simulink model "ATOM_simple_planning_simulator"  (R2026a)
settings: Solver=ode4  StopTime=100  FixedStep=0.01
StopFcn:
  | % Put every new figure in the same MATLAB Figures window as a docked tab.
  | set(groot, 'defaultFigureWindowStyle', 'docked');
  | 
  | if exist('costmap_active', 'var') && ...
  |     exist('vehicle', 'var') && ...
  |     exist('parking_path', 'var') && ...
  |     ~isempty(parking_path)
  | 
  |      plotPlan(costmap_active, vehicle, parking_path);
  | 
  |  else
  | 
  |      warning('No valid parking path is available for plotting.');
  | 
  |  end
  | 
  |  PlotControllerReferences( ...
  |      out.controller_reference_log);
  | 
  |  PlotControllerTracking( ...
  |      out.controller_tracking_log);
  | 
model workspace (MAT data in the model file):
  vehicle : object (value not decoded)
symbols that are objects in the model workspace (value not decoded): vehicle
undefined symbols (not defined in the file): delta_f_LUT, gain4WS_LUT, k_ref_LUT, kappa_gain_BP, Ki, Kp, lateral, longitudinal, planning_validator, rr_gain_BP, rr_LUT, stanley, velocity_smoother
libraries: slpidlib x1
(part 3 of 8)

== matlab function ATOM_simple_planning_simulator/time_parameterization2/Time parameterization ==
  data: trajectory_in input Bus: TrajectoryDataBus size=1; reference_out output Bus: ParkingReferenceBus size=1; steer_rate_limit input
function reference_out = timeParameterization( ...
    trajectory_in,steer_rate_limit)
%#codegen
%
% Convert the 100-point spatial parking trajectory into a nominal
% time-parameterized reference trajectory.

N = 100;

%% Extract the smoothed trajectory

x_ref = trajectory_in.pose.position.x;
y_ref = trajectory_in.pose.position.y;

qz = trajectory_in.pose.orientation.qz;
qw = trajectory_in.pose.orientation.qw;

v_ref = trajectory_in.longitudinal_velocity_mps;
a_ref = trajectory_in.acceleration_mps2;

df_plan = trajectory_in.front_wheel_angle_rad;
dr_plan = trajectory_in.rear_wheel_angle_rad;

rear_angle = trajectory_in.rear_wheel_angle_rad;

%% Convert quaternion to continuous body-heading reference

psi_ref = zeros(N,1);

psi_ref(1) = 2.0*atan2(qz(1),qw(1));

for k = 2:N

    raw_heading = 2.0*atan2(qz(k),qw(k));

    heading_change = raw_heading-psi_ref(k-1);

    psi_ref(k) = ...
        raw_heading-2.0*pi*round(heading_change/(2.0*pi));
end

%% Calculate distance and nominal time

s_ref = zeros(N,1);
t_ref = zeros(N,1);

for k = 1:N-1

    dx = x_ref(k+1)-x_ref(k);
    dy = y_ref(k+1)-y_ref(k);

    ds = hypot(dx,dy);

    s_ref(k+1) = s_ref(k)+ds;

    % Convert signed body-longitudinal velocity to positive rear-axle
    % path speed.
    path_speed_current = ...
        abs(v_ref(k))/max(cos(rear_angle(k)),0.1);

    path_speed_next = ...
        abs(v_ref(k+1))/max(cos(rear_angle(k+1)),0.1);

    speed_sum = path_speed_current+path_speed_next;

    if ds <= 1e-9

        dt = 0.0;

    elseif speed_sum > 1e-6

        % ds = 0.5*(v_current+v_next)*dt
        dt = 2.0*ds/speed_sum;

    else

        % Protect against an interval whose two endpoint speeds are zero.
        fallback_path_speed = 0.05;

        dt = ds/fallback_path_speed;
    end

    t_ref(k+1) = t_ref(k)+dt;
end
N = numel(t_ref);

df_nom = zeros(size(df_plan));
dr_nom = zeros(size(dr_plan));

% Start from the planner's first steering configuration.
df_nom(1) = df_plan(1);
dr_nom(1) = dr_plan(1);

for i = 2:N

    dt = max(t_ref(i)-t_ref(i-1),0.0);
    maximum_change = steer_rate_limit*dt;

    front_difference = df_plan(i)-df_nom(i-1);
    rear_difference  = dr_plan(i)-dr_nom(i-1);

    front_change = max( ...
        -maximum_change, ...
        min(maximum_change,front_difference));

    rear_change = max( ...
        -maximum_change, ...
        min(maximum_change,rear_difference));

    df_nom(i) = df_nom(i-1)+front_change;
    dr_nom(i) = dr_nom(i-1)+rear_change;

end

reference_out.t_ref   = t_ref;
reference_out.s_ref   = s_ref;
reference_out.x_ref   = x_ref;
reference_out.y_ref   = y_ref;
reference_out.psi_ref = psi_ref;
reference_out.v_ref   = v_ref;
reference_out.a_ref   = a_ref;
% Temporary pass-through. The next step will make these rate-feasible.
reference_out.df_nom = df_nom;
reference_out.dr_nom = dr_nom;
end

== matlab function ATOM_simple_planning_simulator/Plot demanded trajectory ==
  data: traj input
function plotTrajectory(traj)

persistent hTraj hArrow


x = traj.pose.position.x;
y = traj.pose.position.y;

yaw = zeros(length(x),1);


for i=1:length(x)

    yaw(i)=2*atan2(...
        traj.pose.orientation.qz(i),...
        traj.pose.orientation.qw(i));

end


if isempty(hTraj)

    figure(2)
    clf
    hold on
    grid on
    axis equal

    hTraj=plot(x,y,'b','LineWidth',2);


    step=5;

    hArrow=quiver(...
        x(1:step:end),...
        y(1:step:end),...
        cos(yaw(1:step:end)),...
        sin(yaw(1:step:end)),...
        0.5,...
        'r');

else

    set(hTraj,...
        'XData',x,...
        'YData',y);

end


drawnow limitrate

end

== matlab function ATOM_simple_planning_simulator/velocity_smoother_node/ApplySteeringRateLimit - velocity_smoother_node/ApplyPreProcess ==
  data: input input Bus: TrajectoryDataBus; use_resempling input boolean; output output Bus: TrajectoryDataBus; points_interval input double
function output = applyPreProcess(input, use_resempling, points_interval)

% ApplyPreProcess
%
% This function reproduces the first stage of Autoware
% SmootherBase::applyPreProcess().
%
% In Autoware, when resampling is enabled, the input trajectory
% is interpolated with a constant spatial interval.
%
% In this Simulink implementation the resampling stage is omitted
% (use_resempling == false)
% The original trajectory points are directly forwarded to the next block.
%

output = input;

end

== matlab function ATOM_simple_planning_simulator/velocity_smoother_node/ApplySteeringRateLimit - velocity_smoother_node/Step1: Calculate curvature assuming the trajectory points interval is constant./CalcTrajectoryCurvature ==
  data: trajectory input Bus: TrajectoryDataBus; curvature output; idx_dist input
function curvature = ComputeTrajectoryCurvature( ...
    trajectory, ...
    idx_dist)

% ComputeTrajectoryCurvature
%
% Computes the geometric curvature of a trajectory using a three-point
% circle fitting method.
%
% This function reproduces the behavior of:
%
% autoware_motion_utils::calcTrajectoryCurvatureFrom3Points()
%
% used inside:
%
% autoware_velocity_smoother
%
% In the original Autoware implementation, the curvature computation:
%
%   curvature = calc_curvature(p0,p1,p2)
%
% is protected by a C++ try/catch block. If the circle fitting fails
% (for example due to degenerate geometry), Autoware keeps the previous
% curvature value.
%
% MATLAB/Simulink code generation does not support try/catch constructs.
% Therefore this implementation assumes that calc_curvature() is robust
% and handles degenerate cases internally.
%
% Inputs
% -------
% trajectory : struct
%
%   MATLAB representation of Autoware TrajectoryPoints.
%
%   Autoware source:
%
%   autoware_motion_utils/src/trajectory/conversion.cpp
%
%   converts:
%
%       autoware_planning_msgs::msg::Trajectory
%
%   into:
%
%       std::vector<autoware_planning_msgs::msg::TrajectoryPoint>
%
%   via:
%
    % std::vector<autoware_planning_msgs::msg::TrajectoryPoint> convertToTrajectoryPointArray(
    % const autoware_planning_msgs::msg::Trajectory & trajectory)
    % {
    %     std::vector<autoware_planning_msgs::msg::TrajectoryPoint> output(trajectory.points.size());
    %     std::copy(trajectory.points.begin(), trajectory.points.end(), output.begin());
    %     return output;
    % }
%
%
%
%   Each trajectory point contains:
%
%       geometry_msgs/msg/Point pose.position
%
%   with:
%
%       x, y, z
%
%   MATLAB representation:
%
%       trajectory.pose.position.x
%       trajectory.pose.position.y
%       trajectory.pose.position.z
%
%
% idx_dist : scalar
%
%   Number of trajectory samples used as offset for the three-point
%   curvature estimation.
%
%   In Autoware:
%
%       idx_dist =
%       max(floor(curvature_calculation_distance / points_interval),1)
%
%
% Output
% -------
% curvature : Nx1 vector
%
%   Estimated trajectory curvature [1/m].

num_points = length(trajectory.pose.position.x);


%% Not enough trajectory points

% Autoware:
%
% if (trajectory.size() < 3)
% {
%     return vector filled with zeros;
% }

if num_points < 3
    curvature = zeros(num_points,1);
    return;
end


%% Limit idx_dist according to trajectory size

% Autoware:
%
% max_idx_dist =
% floor((trajectory.size()-1)/2)
%
% idx_dist =
% max(1,min(idx_dist,max_idx_dist))

max_idx_dist = floor((num_points-1)/2);

idx_dist = max(1,min(idx_dist,max_idx_dist));


%% Initialize curvature vector

% Autoware:
%
% std::vector<double> k_arr(trajectory.size(),0.0);

curvature = zeros(num_points,1);


%% Three-point curvature estimation

% Autoware:
%
% for (size_t i = 1; i + 1 < trajectory.size(); i++)

% MATLAB indexing:
%
% i = 2 ... N-1

for i = 2:num_points-1


    % Select the three points:
    %
    % p0 : idx_dist samples before
    % p1 : current trajectory point
    % p2 : idx_dist samples after
    %
    % Equivalent to Autoware:
    %
    % p0 = get_point(
    %       trajectory.at(i - min(idx_dist,i)))
    %
    % p1 = get_point(
    %       trajectory.at(i))
    %
    % p2 = get_point(
    %       trajectory.at(
    %       i + min(idx_dist,size-i-1)))


    idx_prev = i - min(idx_dist,i-1);

    idx_curr = i;

    idx_next = i + min(idx_dist,num_points-i);


    % geometry_msgs/msg/Point:
    %
    % float64 x
    % float64 y
    % float64 z

    p0 = [
        trajectory.pose.position.x(idx_prev), ...
        trajectory.pose.position.y(idx_prev), ...
        trajectory.pose.position.z(idx_prev)
        ];

    p1 = [
        trajectory.pose.position.x(idx_curr), ...
        trajectory.pose.position.y(idx_curr), ...
        trajectory.pose.position.z(idx_curr)
        ];

    p2 = [
        trajectory.pose.position.x(idx_next), ...
        trajectory.pose.position.y(idx_next), ...
        trajectory.pose.position.z(idx_next)
        ];


    %% Compute curvature

    % Autoware:
    %
    % try
    % {
    %     curvature = calc_curvature(p0,p1,p2);
    % }
    %
    % catch(...)
    % {
    %     curvature = previous curvature;
    % }
    %
    % try/catch removed because unsupported by Simulink Coder.

    curvature(i) = calc_curvature(p0,p1,p2);


end


%% Boundary curvature completion

% Autoware:
%
% k_arr.at(0) = k_arr.at(1);
% k_arr.back() = k_arr.at(size-2);

curvature(1) = curvature(2);

curvature(end) = curvature(end-1);


end

== matlab function ATOM_simple_planning_simulator/velocity_smoother_node/ApplySteeringRateLimit - velocity_smoother_node/Step4: Limit velocity by steer rate./ApplySteeringRateVelocityLimit ==
  data: steer_rate_velocity_ratio_limits input; curvature input; steer_rate_ratio input; curvature_threshold input; min_curve_velocity input; velocity_thresholds input; steering_angle_rate_limits input; trajectory input Bus: TrajectoryDataBus; trajectory output
function trajectory = ApplySteeringRateVelocityLimit( ...
    steer_rate_velocity_ratio_limits, ...
    curvature, ...
    steer_rate_ratio, ...
    curvature_threshold, ...
    min_curve_velocity, ...
    velocity_thresholds, ...
    steering_angle_rate_limits, ...
    trajectory)

% ApplySteeringRateVelocityLimit
%
% Applies the steering-rate velocity constraint to the trajectory.
%
% Equivalent to Step 4 of:
%
%   SmootherBase::applySteeringRateLimit()
%
% in Autoware.
%
%
% The steering rate itself does not directly modify the steering angles.
% Instead, it generates a local maximum admissible velocity.
%
% Whenever the current trajectory speed exceeds this limit,
% the trajectory longitudinal velocity is reduced.
%
%
% This algorithm is identical for both 2WS and 4WS.
%
% The only difference is how steer_rate_ratio has been computed.
%
%
% In C++, the following reference:
%
%   auto & velocity =
%       output.at(i+k).longitudinal_velocity_mps;
%
% directly modifies the trajectory.
%
% MATLAB has no equivalent reference semantics, therefore the trajectory
% structure is explicitly updated.



N = length(trajectory.longitudinal_velocity_mps);


for i = 1:N-1

    %% Ignore almost straight segments

    if abs(curvature(i)) < curvature_threshold
        continue
    end


    %% Mean velocity

    mean_velocity = ...
        ( ...
        trajectory.longitudinal_velocity_mps(i) + ...
        trajectory.longitudinal_velocity_mps(i+1) ...
        ) / 2;


    %% Local steering-rate velocity limit

    local_velocity_limit = ...
        ComputeVelocityLimitFromSteerRate( ...
        steer_rate_ratio(i), ...
        steer_rate_velocity_ratio_limits, ...
        velocity_thresholds, ...
        steering_angle_rate_limits);

    %% If the following condition is true, do nothing and pass to the next iteration

    if mean_velocity < local_velocity_limit
        continue
    end


    %% Update the two neighbouring trajectory points

    % Equivalent in C++ to:
    % for (size_t k = 0; k < 2; k++) {
    %     auto & velocity = output.at(i+k).longitudinal_velocity_mps;
    % 
    %     const float target_velocity =
    %     std::max(
    %     min_curve_velocity,
    %     std::min(
    %     local_velocity_limit,
    %     velocity * (local_velocity_limit / mean_vel)));
    % 
    %     velocity = std::min(velocity,target_velocity);
    %     }

    for k = 0:1

        idx = i + k;

        velocity = ...
            trajectory.longitudinal_velocity_mps(idx);


        target_velocity = max( ...
            min_curve_velocity, ...
            min( ...
                local_velocity_limit, ...
                velocity * ...
                (local_velocity_limit / mean_velocity)));


        trajectory.longitudinal_velocity_mps(idx) = ...
            min(velocity, target_velocity);

    end

end

end

== matlab function ATOM_simple_planning_simulator/velocity_smoother_node/ApplySteeringRateLimit - velocity_smoother_node/Step2: Calculate steer rate for each trajectory point/ComputeSteeringRate4WS ==
  data: trajectory input Bus: TrajectoryDataBus; curvature input; veh input; steer_rate_velocity_ratio_arr output; points_interval input; output output Bus: TrajectoryDataBus; k_ref_LUT input; rr_LUT input; delta_f_LUT input
function [steer_rate_velocity_ratio_arr, output] = ComputeSteeringRateAngle4WS(trajectory, ...
    curvature, veh, ...
    points_interval, ...
    k_ref_LUT, rr_LUT, delta_f_LUT)


% ComputeSteeringRateAngle4WS
%
% Computes steering angle rate ratio for 4WS.
%
% Equivalent to Autoware:
%
% steer_rate_velocity_ratio_arr
%
%
% The returned value represents:
%
%       steering_angle_difference / distance
%
%
% For 4WS:
%
% front and rear steering rates are computed.
%
% The maximum steering variation is used as constraint.


N = length(curvature);

rr = zeros(N,1);
front_angle = zeros(N,1);
rear_angle  = zeros(N,1);


%% Compute steering angles

for i = 1:N
    
    if curvature(i) > max(k_ref_LUT)
        rr(i) = -1;
        front_angle(i) = 0.7;
        rear_angle(i) = -0.7;
    else                                                         % Modified for 4WS
        rr(i) = interp1(k_ref_LUT, rr_LUT, curvature(i));
        front_angle(i) = interp1(k_ref_LUT, delta_f_LUT, curvature(i));
        rear_angle(i) = rr(i) * front_angle(i);      
    end
end

% This is a collateral effect of (&) in C++ when (considering in original
% Autoware):
%
% auto & steer_front = output.at(i + 1).front_wheel_angle_rad;
% auto & steer_back = output.at(i).front_wheel_angle_rad;
% 
% // calculate the just 2 steering angle
% steer_front = std::atan(base_param_.wheel_base * curvature_v.at(i + 1));
% steer_back = std::atan(base_param_.wheel_base * curvature_v.at(i));
% Indeed, updating steer_front we popolate also output.at(i + 1).front_wheel_angle_rad, 
% and so the output topic is populated (but it's just a collateral effect, front_wheel_angle_rad 
% and rear_wheel_angle_rad contents are not important for Control module.

trajectory.front_wheel_angle_rad = front_angle;
trajectory.rear_wheel_angle_rad  = rear_angle;

%% Compute steering rate

steer_rate_velocity_ratio_arr = zeros(N,1);


for i = 1:N-1


    % auto & steer_front = output.at(i + 1).front_wheel_angle_rad;
    % auto & steer_back = output.at(i).front_wheel_angle_rad;
    % const auto steering_diff = std::fabs(steer_front - steer_back);
    front_diff = abs( ...
        front_angle(i+1)-front_angle(i));


    rear_diff = abs( ...
        rear_angle(i+1)-rear_angle(i));


    steering_diff = max( ...                                    % Modified for 4WS --> conservative solution
        front_diff,...
        rear_diff);

    % eps avoids division by zero:
    eps = 2.220446049250313e-16;

    steer_rate_velocity_ratio_arr(i)= ...
        steering_diff/(points_interval+eps);


end


steer_rate_velocity_ratio_arr(end)= ...
    steer_rate_velocity_ratio_arr(end-1);


% Output topic now presents front_wheel_angle_rad and rear_wheel_angle_rad
% populated
output = trajectory;


end

== matlab function ATOM_simple_planning_simulator/velocity_smoother_node/ApplySteeringRateLimit - velocity_smoother_node/Step3: Remove noise by mean filter/MeanFilterSteeringRateRato ==
  data: steer_rate_ratio input; steer_rate_velocity_ratio_arr output
function steer_rate_velocity_ratio_arr = MeanFilterSteeringRateRatio( ...
    steer_rate_ratio)

% MeanFilterSteeringRateRatio
%
% Applies the same moving-average filter used by Autoware on the steering
% rate ratio.
%
% Equivalent to Step 3 inside:
%
%   SmootherBase::applySteeringRateLimit()
%
% in:
%
%   autoware_velocity_smoother
%
%
% Original C++ implementation:
%
% for (size_t i = 1; i < steer_rate_velocity_ratio_arr.size() - 1; i++) {
%
%   steer_rate_velocity_ratio_arr.at(i) =
%     (steer_rate_velocity_ratio_arr.at(i-1) +
%      steer_rate_velocity_ratio_arr.at(i)   +
%      steer_rate_velocity_ratio_arr.at(i+1))
%      / 3.0;
%
% }
%
%
% Notes
% -----
%
% The filter is performed in-place, exactly as in Autoware.
%
% Consequently, when computing sample i, the previous sample
% (i-1) has already been filtered, while the next sample (i+1)
% is still the original one.
%
% This behaviour is intentionally preserved to remain identical
% to the C++ implementation.


N = length(steer_rate_ratio);

steer_rate_velocity_ratio_arr = zeros(N,1);

for i = 2:N-1

    steer_rate_velocity_ratio_arr(i) = ...
        ( ...
        steer_rate_ratio(i-1) + ...
        steer_rate_ratio(i)   + ...
        steer_rate_ratio(i+1) ...
        ) / 3.0;

end


end

== matlab function ATOM_simple_planning_simulator/velocity_smoother_node/ApplySteeringRateLimit - velocity_smoother_node/ComputePointsInterval ==
  data: input_points_interval input; vel_smoother input; use_resampling input; points_interval output
function points_interval = computePointsInterval(input_points_interval, ...
    vel_smoother, use_resampling)

% Compute the trajectory points interval used for preprocessing.
%
% If resampling is enabled, a constant spatial interval is imposed.
% Otherwise, the original trajectory point spacing is preserved.

sample_ds = vel_smoother(3,1);

if use_resampling

    points_interval = sample_ds;

else

    points_interval = input_points_interval;

end

end

== matlab function ATOM_simple_planning_simulator/velocity_smoother_node/ApplySteeringRateLimit - velocity_smoother_node/ComputeIdxDist ==
  data: points_interval input; idx_dist output; vel_smoother input
function idx_dist = ComputeIdxDist( ...
    points_interval, ...
    vel_smoother)

% ComputeIdxDist
%
% Computes the point offset used for trajectory curvature estimation.
%
% The curvature is evaluated using three trajectory points separated by a
% fixed physical distance. Since the trajectory is sampled with a constant
% spatial interval (points_interval), this function converts the desired
% curvature calculation distance into the corresponding point index offset.
%
% In other words, idx_dist represents the number of trajectory points
% corresponding to the specified curvature calculation distance.
%
% Equivalent to the Autoware implementation:
%
% idx_dist = max(int(curvature_calculation_distance / points_interval), 1);

curvature_calculation_distance = vel_smoother(1);

idx_dist = max( ...
    floor(curvature_calculation_distance / points_interval), ...
    1);

== matlab function ATOM_simple_planning_simulator/velocity_smoother_node/ApplySteeringRateLimit - velocity_smoother_node/PlotTrajectoryCurvature ==
  data: trajectory input; curvature input
function PlotTrajectoryCurvature(trajectory, curvature)

% PlotTrajectoryCurvature
%
% Visualizes the trajectory curvature computed by:
%
%   ComputeTrajectoryCurvature()
%
% Equivalent to inspecting:
%
%   std::vector<double> k_arr
%
% generated inside:
%
%   autoware_motion_utils::calcTrajectoryCurvatureFrom3Points()
%
%
% Inputs
% -------
%
% trajectory:
%   MATLAB representation of Autoware TrajectoryPoints:
%
%       trajectory.pose.position.x
%       trajectory.pose.position.y
%
%
% curvature:
%   Nx1 signed curvature vector [1/m].
%
%   Positive curvature  -> left turn
%   Negative curvature  -> right turn


persistent hCurvature
persistent hTraj


%% Extract trajectory position

x = trajectory.pose.position.x;
y = trajectory.pose.position.y;


%% Check dimensions

if length(curvature) ~= length(x)

    error("Curvature vector length does not match trajectory length.");

end


%% Curvature profile

if isempty(hCurvature) 

    figure(3)
    clf

    hold on
    grid on

    hCurvature = plot( ...
        curvature, ...
        'LineWidth',1.5);


    xlabel("Trajectory point index");
    ylabel("Curvature [1/m]");

    title("Curvature profile");


else

    set(hCurvature,...
        'YData',curvature);

end



%% XY trajectory colored by curvature

if isempty(hTraj) 

    figure(4)
    clf

    hold on
    grid on
    axis equal


    hTraj = scatter( ...
        x, ...
        y, ...
        25, ...
        curvature, ...
        'filled');


    xlabel("x [m]");
    ylabel("y [m]");

    title("Trajectory curvature map");


    cb = colorbar;
    ylabel(cb,'Curvature [1/m]');


else

    set(hTraj,...
        'XData',x,...
        'YData',y,...
        'CData',curvature);

end


drawnow limitrate


end

== matlab function ATOM_simple_planning_simulator/velocity_smoother_node/ApplySteeringRateLimit - velocity_smoother_node/ComputeSteerRateVelocityRatioLimits ==
  data: velocity_thresholds input; steer_rate_velocity_ratio_limits output; steering_angle_rate_limits input
function steer_rate_velocity_ratio_limits = ...
    ComputeSteerRateVelocityRatioLimits( ...
    velocity_thresholds, ...
    steering_angle_rate_limits)

% ComputeSteerRateVelocityRatioLimits
%
% MATLAB equivalent of:
%
%   SmootherBase::computeSteerRateVelocityRatioLimits()
%
% in Autoware.
%
% It computes the steering-rate / velocity ratio limits used later by
% ComputeVelocityLimitFromSteerRate().
%
%
% Equivalent C++:
%
% return computeRatioLimits<double>(
%     velocity_thresholds,
%     steering_angle_rate_limits,
%     compute_steer_rate_ratio);
%
%
% Inputs
% -------
%
% velocity_thresholds
%       Velocity breakpoints [m/s]
%
% steering_angle_rate_limits
%       Maximum steering rate [deg/s]
%
%
% Output
% ------
%
% steer_rate_velocity_ratio_limits
%
% Nx2 matrix equivalent to:
%
% std::vector<std::pair<double,double>>
%
% Each row contains:
%
%   [ratio_lower , ratio_upper]
%
% corresponding to one velocity interval.


epsilon = 1e-5;

N = length(velocity_thresholds);

steer_rate_velocity_ratio_limits = zeros(N+1,2);


%% Compute ratio limits

for i = 1:N

    rate_deg = steering_angle_rate_limits(i);

    vi = velocity_thresholds(i);

    if i == 1
        vi_prev = 0.0;
    else
        vi_prev = velocity_thresholds(i-1);
    end

    steer_rate_velocity_ratio_limits(i,1) = ...
        deg2rad(rate_deg)/(vi_prev + epsilon);

    steer_rate_velocity_ratio_limits(i,2) = ...
        deg2rad(rate_deg)/(vi + epsilon);

end


%% Last interval

v_max = velocity_thresholds(end);

steer_rate_velocity_ratio_limits(end,1) = ...
    deg2rad(steering_angle_rate_limits(end)) / ...
    (v_max + epsilon);

steer_rate_velocity_ratio_limits(end,2) = 0.0;

end

== matlab function ATOM_simple_planning_simulator/velocity_smoother_node/MATLAB Function ==
  data: trajectory_input input; trajectory_output input; curvature input
function PlotSteeringRateVelocityLimit( ...
    trajectory_input, ...
    trajectory_output, ...
    curvature)

% PlotSteeringRateVelocityLimit
%
% Visualizes the velocity modification produced by the steering-rate
% velocity constraint.
%
% Equivalent to inspecting the difference between:
%
%   input.longitudinal_velocity_mps
%
% and:
%
%   output.longitudinal_velocity_mps
%
% after:
%
%   SmootherBase::applySteeringRateLimit()
%
% in Autoware.
%
%
% The steering-rate filter does not modify the trajectory geometry.
% It only reduces longitudinal velocity where the steering rate
% constraint is violated.
%
%
% Inputs
% -------
%
% trajectory_input:
%       Trajectory before ApplySteeringRateVelocityLimit()
%
%       Required fields:
%           trajectory.longitudinal_velocity_mps
%
%
% trajectory_output:
%       Trajectory after ApplySteeringRateVelocityLimit()
%
%       Required fields:
%           trajectory.longitudinal_velocity_mps
%
%
% curvature:
%       trajectory curvature [1/m]
%
%       Used only for visualization of curved regions.
%
%
% Output
% -------
%
% None
%
% Generates diagnostic plots:
%
%   - velocity before/after steering-rate constraint
%   - velocity reduction
%   - curvature profile


%% Extract velocities

vel_in = trajectory_input.longitudinal_velocity_mps;
vel_out = trajectory_output.longitudinal_velocity_mps;


N = length(vel_in);


if length(vel_out) ~= N
    error("Input and output trajectories have different lengths.");
end


%% Velocity variation

velocity_delta = vel_out - vel_in;


%% Plot velocity profile

persistent hVelIn hVelOut hCurvature hVelDelta1 hVelDelta2


if isempty(hVelIn)

    figure(5)
    hold on
    grid on

    hVelIn = plot( ...
        vel_in,...
        'LineWidth',1.5,...
        'DisplayName',"Input velocity");
    
    hVelOut = plot( ...
        vel_out,...
        '--',...
        'LineWidth',1.5,...
        'DisplayName',"After steering-rate limit");


    xlabel("Trajectory point index");
    ylabel("Longitudinal velocity [m/s]");
    
    title("Steering-rate velocity limitation");
    
    legend("Location","best");

else
    
    set(hVelIn, ...
        'YData', vel_in);
    
    set(hVelOut, ...
        'YData', vel_out);
end

%% Plot velocity reduction


if isempty(hVelDelta1)

    figure(6)
    hold on
    grid on

    hVelDelta1 = plot( ...
        velocity_delta,...
        'LineWidth',1.5);
    
    
    yline(0);
    
    
    xlabel("Trajectory point index");
    ylabel("\Delta velocity [m/s]");
    
    
    title("Velocity modification due to steering-rate constraint");

else

    set(hVelDelta1, ...
        'YData', velocity_delta);


end

drawnow limitrate

end

== matlab function ATOM_simple_planning_simulator/Lane Follower Scenario/Demanded trajectory generation: Sinusoid 50m wavelength/Trajectory Generator: sinusoid ==
  data: x output; y output; z output; qx output; qy output; qz output; qw output; longitudinal_velocity_mps output; lateral_velocity_mps output; acceleration_mps2 output; heading_rate_rps output; front_wheel_angle_rad output; rear_wheel_angle_rad output
function [x,y,z,qx,qy,qz,qw,...
    longitudinal_velocity_mps,...
    lateral_velocity_mps,...
    acceleration_mps2,...
    heading_rate_rps,...
    front_wheel_angle_rad,...
    rear_wheel_angle_rad] = trajectoryGenerator

N = 100;

L = 100;                % trajectory length [m]
A = 5;                  % sinusoid amplitude [m]

x = linspace(0,L,N)';
y = A*sin(2*pi*x/50);      % wavelength = 50 m

z = zeros(N,1);

qx = zeros(N,1);
qy = zeros(N,1);
qz = zeros(N,1);
qw = zeros(N,1);

longitudinal_velocity_mps = (8/3.6)*ones(N,1);

lateral_velocity_mps = zeros(N,1);
acceleration_mps2    = zeros(N,1);
heading_rate_rps     = zeros(N,1);

front_wheel_angle_rad = zeros(N,1);
rear_wheel_angle_rad  = zeros(N,1);

%% Orientation

dy = gradient(y,x);

yaw = atan(dy);

qz = sin(yaw/2);
qw = cos(yaw/2);

end

== matlab function ATOM_simple_planning_simulator/Lane Follower Scenario/Demanded trajectory generation: 90° left turn/Trajectory Generator: 90° left turn ==
  data: x output; y output; z output; qx output; qy output; qz output; qw output; longitudinal_velocity_mps output; lateral_velocity_mps output; acceleration_mps2 output; heading_rate_rps output; front_wheel_angle_rad output; rear_wheel_angle_rad output
function [x,y,z,qx,qy,qz,qw,...
          longitudinal_velocity_mps,...
          lateral_velocity_mps,...
          acceleration_mps2,...
          heading_rate_rps,...
          front_wheel_angle_rad,...
          rear_wheel_angle_rad] = trajectoryGenerator

N = 100;

%% Geometry

R = 10;              % curve radius [m]

N1 = 30;            % first straight
N2 = 40;            % circular arc
N3 = 30;            % second straight


%% Allocate outputs

x = zeros(N,1);
y = zeros(N,1);
z = zeros(N,1);

qx = zeros(N,1);
qy = zeros(N,1);
qz = zeros(N,1);
qw = zeros(N,1);

longitudinal_velocity_mps = (15/3.6)*ones(N,1);

lateral_velocity_mps = zeros(N,1);
acceleration_mps2 = zeros(N,1);
heading_rate_rps = zeros(N,1);

front_wheel_angle_rad = zeros(N,1);
rear_wheel_angle_rad = zeros(N,1);


%% ------------------------------------------------------------------------
%% First straight
%% ------------------------------------------------------------------------

L1 = 15;

for i = 1:N1

    t = (i-1)/(N1-1);

    x(i) = t*L1;
    y(i) = 0;

    yaw = 0;

    qz(i) = sin(yaw/2);
    qw(i) = cos(yaw/2);

end


%% ------------------------------------------------------------------------
%% Circular arc (90 deg)
%% ------------------------------------------------------------------------

center_x = L1;
center_y = R;

theta = linspace(-pi/2,0,N2);

for k = 1:N2

    i = N1+k;

    x(i) = center_x + R*cos(theta(k));
    y(i) = center_y + R*sin(theta(k));

    yaw = theta(k)+pi/2;

    qz(i) = sin(yaw/2);
    qw(i) = cos(yaw/2);

end


%% ------------------------------------------------------------------------
%% Second straight
%% ------------------------------------------------------------------------

L2 = 15;

x0 = x(N1+N2);
y0 = y(N1+N2);

for k = 1:N3

    i = N1+N2+k;

    t = k/(N3);

    x(i) = x0;
    y(i) = y0 + t*L2;

    yaw = pi/2;

    qz(i) = sin(yaw/2);
    qw(i) = cos(yaw/2);

end

end

== matlab function ATOM_simple_planning_simulator/trajectory_checker plugin - planning_validator_node/check_valid_steering/calcMaxSteeringAngles/calcSteeringAngles/calcCurvature ==
  data: trajectory input Bus: TrajectoryDataBus; curvature_vector output
function curvature_vector = ComputeTrajectoryCurvaturePlanningValidator(trajectory)

% ComputeTrajectoryCurvaturePlanningValidator
%
% Computes the trajectory curvature exactly as performed by the
% Autoware Planning Validator.
%
% Unlike VelocitySmoother, this implementation does NOT use idx_dist.
%
% Instead, for each trajectory point it searches the first previous and
% next trajectory points located at least:
%
%       curvature_distance = 1.0 [m]
%
% away along the trajectory arc length.
%
% The three selected points are then used by calcCurvature().
%
% This implementation reproduces:
%
% trajectory_checker_utils::calcCurvature()
%
% used inside:
%
% planning_validator
%
%
% Inputs
% -------
%
% trajectory
%
% MATLAB representation of Trajectory.
%
%
% Output
% -------
%
% curvature
%
% Nx1 curvature vector [1/m].

num_points = length(trajectory.pose.position.x);

curvature = zeros(num_points,1);

%% Need at least three points

if num_points < 3
    return
end

%% Arc-length computation

arc_length = zeros(num_points,1);

for i = 2:num_points

    dx = trajectory.pose.position.x(i) - ...
         trajectory.pose.position.x(i-1);

    dy = trajectory.pose.position.y(i) - ...
         trajectory.pose.position.y(i-1);

    ds = hypot(dx,dy);

    arc_length(i) = arc_length(i-1) + ds;

end

%% Curvature computation

curvature_distance = 1.0;      % [m]

first_distant_index = 0;
last_distant_index  = num_points;

for i = 2:num_points-1

    %% Search previous point

    idx_prev = 1;

    for j = i-1:-1:2

        if (arc_length(i)-arc_length(j)) > curvature_distance

            if first_distant_index == 0
                first_distant_index = i;
            end

            idx_prev = j;
            break

        end

    end

    %% Search next point

    idx_next = num_points;

    for j = i+1:num_points-1

        if (arc_length(j)-arc_length(i)) > curvature_distance

            last_distant_index = i;

            idx_next = j;
            break

        end

    end

    %% Extract points

    p1 = [
        trajectory.pose.position.x(idx_prev), ...
        trajectory.pose.position.y(idx_prev), ...
        trajectory.pose.position.z(idx_prev)
        ];

    p2 = [
        trajectory.pose.position.x(i), ...
        trajectory.pose.position.y(i), ...
        trajectory.pose.position.z(i)
        ];

    p3 = [
        trajectory.pose.position.x(idx_next), ...
        trajectory.pose.position.y(idx_next), ...
        trajectory.pose.position.z(idx_next)
        ];

    % In Autoware this call is wrapped inside a try/catch.
    % Since MATLAB code generation does not support exceptions,
    % calcCurvature() is assumed to always return a valid value.
    curvature(i) = calc_curvature(p1,p2,p3);

end

%% Replicate boundary values

% Equivalent to:
%
% for (size_t i = first_distant_index; i > 0; --i)
%   curvature(i-1)=curvature(i);

if first_distant_index > 0

    for i = first_distant_index:-1:2
        curvature(i-1) = curvature(i);
    end

end

% Equivalent to:
%
% for (size_t i = last_distant_index;
%      i < curvature.size()-1;
%      ++i)
%   curvature(i+1)=curvature(i);

if last_distant_index < num_points

    for i = last_distant_index:num_points-1
        curvature(i+1) = curvature(i);
    end

end

curvature_vector = curvature;

end

== matlab function ATOM_simple_planning_simulator/trajectory_checker plugin - planning_validator_node/check_valid_steering/calcMaxSteeringAngles/calcSteeringAngles/steering_vector calculation ==
  data: curvature input; front_steering_vector output; rear_steering_vector output; veh input
function [front_steering_vector, rear_steering_vector] = calcSteeringVector(curvature, veh)

wheel_base = veh(3);
rear_steering_ratio = veh(29);

N = length(curvature);

front_steering_vector = zeros(N,1);
rear_steering_vector  = zeros(N,1);

for i = 1:N

    front_steering_vector(i) = ...
        CalculateFrontSteeringAngle4WS( ...
        curvature(i),...
        wheel_base,...
        rear_steering_ratio);

    rear_steering_vector(i) = rear_steering_ratio*front_steering_vector(i);
    
end
    
end

== matlab function ATOM_simple_planning_simulator/trajectory_checker plugin - planning_validator_node/check_valid_steering/calcMaxSteeringAngles/GetAbsMaxValAndIdx front ==
  data: values input; max_value output; max_index output
function [max_value, max_index] = GetAbsMaxValAndIdx(values)

% GetAbsMaxValAndIdx
%
% Returns the maximum absolute value contained in the input vector and
% its corresponding index.
%
% Equivalent to:
%
% trajectory_checker_utils::getAbsMaxValAndIdx()
%
% in Autoware.
%
% C++ implementation:
%
% std::pair<double, size_t> getAbsMaxValAndIdx(...)
%
% which internally uses:
%
%   std::max_element(...)
%
% with the comparison:
%
%   abs(a) < abs(b)
%
%
% Inputs
% -------
%
% values
%     Nx1 vector.
%
%
% Outputs
% --------
%
% max_value
%     Maximum absolute value contained in the vector.
%
% max_index
%     Index of the element whose absolute value is maximum.
%
% Note
% ----
%
% MATLAB indices are 1-based, whereas the equivalent C++ implementation
% returns a 0-based index.

[max_value, max_index] = max(abs(values));

end

== matlab function ATOM_simple_planning_simulator/trajectory_checker plugin - planning_validator_node/check_valid_steering/calcMaxSteeringAngles/GetAbsMaxValAndIdx rear ==
  data: values input; max_value output; max_index output
function [max_value, max_index] = GetAbsMaxValAndIdx(values)

% GetAbsMaxValAndIdx
%
% Returns the maximum absolute value contained in the input vector and
% its corresponding index.
%
% Equivalent to:
%
% trajectory_checker_utils::getAbsMaxValAndIdx()
%
% in Autoware.
%
% C++ implementation:
%
% std::pair<double, size_t> getAbsMaxValAndIdx(...)
%
% which internally uses:
%
%   std::max_element(...)
%
% with the comparison:
%
%   abs(a) < abs(b)
%
%
% Inputs
% -------
%
% values
%     Nx1 vector.
%
%
% Outputs
% --------
%
% max_value
%     Maximum absolute value contained in the vector.
%
% max_index
%     Index of the element whose absolute value is maximum.
%
% Note
% ----
%
% MATLAB indices are 1-based, whereas the equivalent C++ implementation
% returns a 0-based index.

[max_value, max_index] = max(abs(values));

end

== matlab function ATOM_simple_planning_simulator/trajectory_checker plugin - planning_validator_node/check_valid_steering/calcMaxSteeringAngles/DecideValIdx ==
  data: max_steering output; max_index output; max_front input; idx_front input; max_rear input; idx_rear input
function [max_steering, max_index] = DecideValIdx(max_front, idx_front, ...
                                                  max_rear, idx_rear) 


if max_front >= max_rear

    max_steering = max_front;
    max_index    = idx_front;

else

    max_steering = max_rear;
    max_index    = idx_rear;

end

end

== matlab function ATOM_simple_planning_simulator/trajectory_checker plugin - planning_validator_node/check_valid_steering/CheckValidSteering ==
  data: max_steering input; is_valid_steering output; steering_threshold input
function is_valid_steering  = ...
    CheckValidSteering4WS( ...
    max_steering, steering_threshold)


% CheckValidSteering4WS
%
% Equivalent to:
%
% TrajectoryChecker::check_valid_steering()
%
% Autoware planning_validator
%
%
% The steering angle is NOT taken from:
%
%   trajectory.front_wheel_angle_rad
%   trajectory.rear_wheel_angle_rad
%
% Instead, Autoware recomputes it from trajectory geometry:
%
%   trajectory
%        |
%        v
%   curvature_vector
%        |
%        v
%   steering angle
%
%
% Adapted for 4WS:
%
% curvature =
%
%       (tan(delta_f)-tan(delta_r))/L
%
%
% where:
%
%       delta_r = rear_steering_ratio * delta_f
%
%
% Inputs
% -------
%
% trajectory:
%
%   trajectory.pose.position.x
%   trajectory.pose.position.y
%
%
% wheel_base:
%
%   vehicle wheelbase [m]
%
%
% rear_steering_ratio:
%
%   rear/front steering ratio
%
%
% steering_threshold:
%
%   maximum allowed steering angle [rad]
%
%
%
% Outputs
% --------
%
% is_valid_steering:
%
%   true  -> steering OK
%   false -> steering violation
%
%
% max_steering:
%
%   maximum absolute steering angle [rad]
%
%
% max_index:
%
%   trajectory point where maximum steering occurs
%
%
%

%% ============================================================
% Equivalent to:
%
% if (max_steering > params_.steering.threshold)
%
% =============================================================


if max_steering > steering_threshold

    is_valid_steering = false;

else

    is_valid_steering = true;

end


end

== matlab function ATOM_simple_planning_simulator/trajectory_checker plugin - planning_validator_node/check_valid_steering_rate/CheckValidSteeringRate ==
  data: max_steering_rate input; is_valid_steering_rate output; steering_rate_threshold input
function is_valid_steering_rate  = ...
    CheckValidSteering4WS( ...
    max_steering_rate, steering_rate_threshold)


% CheckValidSteering4WS
%
% Equivalent to:
%
% TrajectoryChecker::check_valid_steering()
%
% Autoware planning_validator
%
%
% The steering angle is NOT taken from:
%
%   trajectory.front_wheel_angle_rad
%   trajectory.rear_wheel_angle_rad
%
% Instead, Autoware recomputes it from trajectory geometry:
%
%   trajectory
%        |
%        v
%   curvature_vector
%        |
%        v
%   steering angle
%
%
% Adapted for 4WS:
%
% curvature =
%
%       (tan(delta_f)-tan(delta_r))/L
%
%
% where:
%
%       delta_r = rear_steering_ratio * delta_f
%
%
% Inputs
% -------
%
% trajectory:
%
%   trajectory.pose.position.x
%   trajectory.pose.position.y
%
%
% wheel_base:
%
%   vehicle wheelbase [m]
%
%
% rear_steering_ratio:
%
%   rear/front steering ratio
%
%
% steering_threshold:
%
%   maximum allowed steering angle [rad]
%
%
%
% Outputs
% --------
%
% is_valid_steering:
%
%   true  -> steering OK
%   false -> steering violation
%
%
% max_steering:
%
%   maximum absolute steering angle [rad]
%
%
% max_index:
%
%   trajectory point where maximum steering occurs
%
%
%

%% ============================================================
% Equivalent to:
%
% if (max_steering > params_.steering.threshold)
%
% =============================================================


if max_steering_rate > steering_rate_threshold

    is_valid_steering_rate = false;

else

    is_valid_steering_rate = true;

end


end

== matlab function ATOM_simple_planning_simulator/trajectory_checker plugin - planning_validator_node/check_valid_steering_rate/calcMaxSteeringRates/DecideValIdx ==
  data: max_steering_rate output; max_index output; max_front input; idx_front input; max_rear input; idx_rear input
function [max_steering_rate, max_index] = DecideValIdx(max_front, idx_front, ...
                                                  max_rear, idx_rear) 


if max_front >= max_rear

    max_steering_rate = max_front;
    max_index    = idx_front;

else

    max_steering_rate = max_rear;
    max_index    = idx_rear;

end

end

== matlab function ATOM_simple_planning_simulator/trajectory_checker plugin - planning_validator_node/check_valid_steering_rate/calcMaxSteeringRates/MATLAB Function ==
  data: trajectory input; max_steering_rate output; steering_vector input; max_index output
function [max_steering_rate, max_index] = ...
    CalcMaxSteeringRate(trajectory, steering_vector)


% CalcMaxSteeringRate
%
% Equivalent to:
%
% trajectory_checker_utils::calcMaxSteeringRates()
%
% in Autoware planning_validator.
%
%
% For 2WS:
%   steering_vector = front steering angle
%
% For 4WS:
%   call this function twice:
%
%   front_rate = CalcMaxSteeringRate(trajectory, front_vector)
%   rear_rate  = CalcMaxSteeringRate(trajectory, rear_vector)
%
% and take:
%
%   max(front_rate,rear_rate)
%
%
% Steering rate:
%
%       d(delta)/dt
%
% where:
%
%       dt = delta_s / velocity
%
%
% Units:
%
% steering_vector : [rad]
% trajectory velocity : [m/s]
% output : [rad/s]


N = length(steering_vector);


if N < 2

    max_steering_rate = 0;
    max_index = 1;

    return

end


max_steering_rate = 0;
max_index = 1;



for i = 1:N-1


    %% Distance between trajectory points

    dx = trajectory.pose.position.x(i+1) - ...
         trajectory.pose.position.x(i);

    dy = trajectory.pose.position.y(i+1) - ...
         trajectory.pose.position.y(i);


    delta_s = sqrt(dx^2 + dy^2);



    %% Mean velocity

    v = 0.5 * ( ...
        trajectory.longitudinal_velocity_mps(i+1) + ...
        trajectory.longitudinal_velocity_mps(i));



    %% Equivalent of:
    %
    % delta_s / max(v,1e-5)
    %
    % in C++

    dt = delta_s / max(v,1e-5);



    %% Steering rate

    steer_rate = ...
        (steering_vector(i+1)-steering_vector(i)) / dt;



    %% Equivalent of takeBigger()

    if abs(steer_rate) > max_steering_rate

        max_steering_rate = abs(steer_rate);

        max_index = i;

    end

end


end

== matlab function ATOM_simple_planning_simulator/trajectory_checker plugin - planning_validator_node/check_valid_steering_rate/calcMaxSteeringRates/MATLAB Function1 ==
  data: trajectory input; max_steering_rate output; steering_vector input; max_index output
function [max_steering_rate, max_index] = ...
    CalcMaxSteeringRate(trajectory, steering_vector)


% CalcMaxSteeringRate
%
% Equivalent to:
%
% trajectory_checker_utils::calcMaxSteeringRates()
%
% in Autoware planning_validator.
%
%
% For 2WS:
%   steering_vector = front steering angle
%
% For 4WS:
%   call this function twice:
%
%   front_rate = CalcMaxSteeringRate(trajectory, front_vector)
%   rear_rate  = CalcMaxSteeringRate(trajectory, rear_vector)
%
% and take:
%
%   max(front_rate,rear_rate)
%
%
% Steering rate:
%
%       d(delta)/dt
%
% where:
%
%       dt = delta_s / velocity
%
%
% Units:
%
% steering_vector : [rad]
% trajectory velocity : [m/s]
% output : [rad/s]


N = length(steering_vector);


if N < 2

    max_steering_rate = 0;
    max_index = 1;

    return

end


max_steering_rate = 0;
max_index = 1;



for i = 1:N-1


    %% Distance between trajectory points

    dx = trajectory.pose.position.x(i+1) - ...
         trajectory.pose.position.x(i);

    dy = trajectory.pose.position.y(i+1) - ...
         trajectory.pose.position.y(i);


    delta_s = sqrt(dx^2 + dy^2);



    %% Mean velocity

    v = 0.5 * ( ...
        trajectory.longitudinal_velocity_mps(i+1) + ...
        trajectory.longitudinal_velocity_mps(i));



    %% Equivalent of:
    %
    % delta_s / max(v,1e-5)
    %
    % in C++

    dt = delta_s / max(v,1e-5);



    %% Steering rate

    steer_rate = ...
        (steering_vector(i+1)-steering_vector(i)) / dt;



    %% Equivalent of takeBigger()

    if abs(steer_rate) > max_steering_rate

        max_steering_rate = abs(steer_rate);

        max_index = i;

    end

end


end

== matlab function ATOM_simple_planning_simulator/trajectory_checker plugin - planning_validator_node/check_valid_steering_rate/calcMaxSteeringRates/calcSteeringAngles/calcCurvature ==
  data: trajectory input Bus: TrajectoryDataBus; curvature_vector output
function curvature_vector = ComputeTrajectoryCurvaturePlanningValidator(trajectory)

% ComputeTrajectoryCurvaturePlanningValidator
%
% Computes the trajectory curvature exactly as performed by the
% Autoware Planning Validator.
%
% Unlike VelocitySmoother, this implementation does NOT use idx_dist.
%
% Instead, for each trajectory point it searches the first previous and
% next trajectory points located at least:
%
%       curvature_distance = 1.0 [m]
%
% away along the trajectory arc length.
%
% The three selected points are then used by calcCurvature().
%
% This implementation reproduces:
%
% trajectory_checker_utils::calcCurvature()
%
% used inside:
%
% planning_validator
%
%
% Inputs
% -------
%
% trajectory
%
% MATLAB representation of Trajectory.
%
%
% Output
% -------
%
% curvature
%
% Nx1 curvature vector [1/m].

num_points = length(trajectory.pose.position.x);

curvature = zeros(num_points,1);

%% Need at least three points

if num_points < 3
    return
end

%% Arc-length computation

arc_length = zeros(num_points,1);

for i = 2:num_points

    dx = trajectory.pose.position.x(i) - ...
         trajectory.pose.position.x(i-1);

    dy = trajectory.pose.position.y(i) - ...
         trajectory.pose.position.y(i-1);

    ds = hypot(dx,dy);

    arc_length(i) = arc_length(i-1) + ds;

end

%% Curvature computation

curvature_distance = 1.0;      % [m]

first_distant_index = 0;
last_distant_index  = num_points;

for i = 2:num_points-1

    %% Search previous point

    idx_prev = 1;

    for j = i-1:-1:2

        if (arc_length(i)-arc_length(j)) > curvature_distance

            if first_distant_index == 0
                first_distant_index = i;
            end

            idx_prev = j;
            break

        end

    end

    %% Search next point

    idx_next = num_points;

    for j = i+1:num_points-1

        if (arc_length(j)-arc_length(i)) > curvature_distance

            last_distant_index = i;

            idx_next = j;
            break

        end

    end

    %% Extract points

    p1 = [
        trajectory.pose.position.x(idx_prev), ...
        trajectory.pose.position.y(idx_prev), ...
        trajectory.pose.position.z(idx_prev)
        ];

    p2 = [
        trajectory.pose.position.x(i), ...
        trajectory.pose.position.y(i), ...
        trajectory.pose.position.z(i)
        ];

    p3 = [
        trajectory.pose.position.x(idx_next), ...
        trajectory.pose.position.y(idx_next), ...
        trajectory.pose.position.z(idx_next)
        ];

    % In Autoware this call is wrapped inside a try/catch.
    % Since MATLAB code generation does not support exceptions,
    % calcCurvature() is assumed to always return a valid value.
    curvature(i) = calc_curvature(p1,p2,p3);

end

%% Replicate boundary values

% Equivalent to:
%
% for (size_t i = first_distant_index; i > 0; --i)
%   curvature(i-1)=curvature(i);

if first_distant_index > 0

    for i = first_distant_index:-1:2
        curvature(i-1) = curvature(i);
    end

end

% Equivalent to:
%
% for (size_t i = last_distant_index;
%      i < curvature.size()-1;
%      ++i)
%   curvature(i+1)=curvature(i);

if last_distant_index < num_points

    for i = last_distant_index:num_points-1
        curvature(i+1) = curvature(i);
    end

end

curvature_vector = curvature;

end
